simulink model "sf_edge_detection_pulse"  (R2025b)
settings: Solver=FixedStepDiscrete  StartTime=0.0  StopTime=8  FixedStep=1  RelTol=1e-3  EnableMultiTasking=on
settings Model: Creator=The MathWorks, Inc.  LastModifiedBy=The MathWorks, Inc.
settings SolverCC: AlgebraicLoopSolver=TrustRegion  MaxZcPerStep=1.0
settings DataIOCC: LimitDataPoints=on  SaveFormat=Array  ReturnWorkspaceOutputs=off
settings OptimizationCC: ReuseModelBlockBuffer=off  ExpressionDepthLimit=2147483647.0  InitFltsAndDblsToZero=on  LifeSpan=inf
settings DebuggingCC: SaveWithParameterizedLinksMsg=none  UnderspecifiedInitializationDetection=Classic  MergeDetectMultiDrivingBlocksExec=none  SignalResolutionControl=TryResolveAllWithWarning  SolverPrmCheckMsg=warning  FcnCallInpInsideContextMsg=warning  UnconnectedInputMsg=warning  UnconnectedOutputMsg=warning  UnconnectedLineMsg=warning  StateNameClashWarn=warning  SFUnexpectedBacktrackingDiag=warning  SFNoUnconditionalDefaultTransitionDiag=warning  SFExecutionAtInitializationDiag=none  ArithmeticOperatorsInVariantConditions=warning
settings HardwareCC: ProdBitPerPointer=32.0  ProdBitPerSizeT=32.0  ProdBitPerPtrDiffT=32.0  ProdLargestAtomicFloat=None  ProdIntDivRoundTo=Undefined  ProdEndianess=Unspecified  ProdWordSize=32.0  ProdHWDeviceType=32-bit Generic
settings ModelReferenceCC: EnableRefExpFcnMdlSchedulingChecks=on  PropagateSignalLabelsOutOfModel=off
settings SFSimCC: SimUseLocalCustomCode=off  SimParseCustomCode=off  CustomCodeUndefinedFunction=UseInterfaceOnly
settings RTWCC: RTWUseLocalCustomCode=off  GPUComputeCapability=3.5  DLArmComputeVersion=19.05
settings CodeAppCC: StateflowObjectComments=on
settings GRTTargetCC: TargetFcnLib=ansi_tfl_tmw.mat  TargetLangStandard=C89/C90 (ANSI)  CombineOutputUpdateFcns=off  GRTInterface=on
settings ConfigComp: CovMetricSettings=dw  CovSaveCumulativeToWorkspaceVar=on  CovSaveSingleToWorkspaceVar=on  CovExternalEMLEnable=off

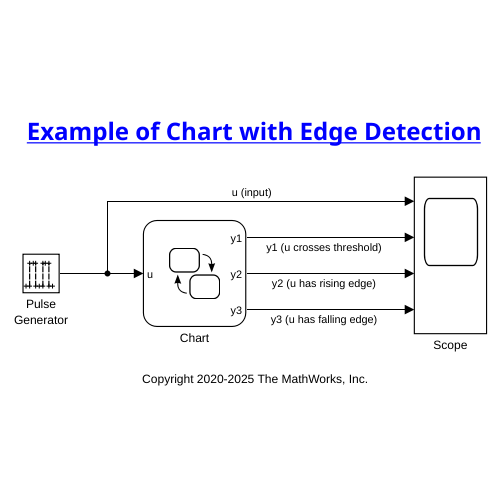
[thumbnail: Simulink's stored preview of the top-level diagram]
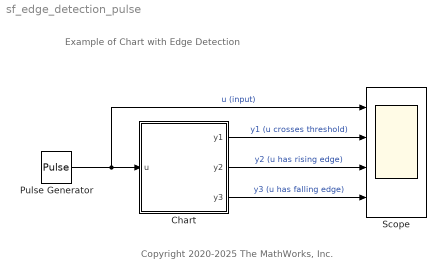
== system sf_edge_detection_pulse ==
  note: Copyright 2020-2025 The MathWorks, Inc.
  note: Example of Chart with Edge Detection
  Chart : Stateflow chart  TreatAsAtomicUnit=on
  Pulse Generator : DiscretePulseGenerator  Amplitude=5  Period=4  PulseWidth=2  PhaseDelay=1
  Scope : Scope  NumInputPorts=4
      settings: ActiveDisplayYMinimum=-0.625  ActiveDisplayYMaximum=5.625
  wires:
  Pulse Generator/1 -> Scope/1, Chart/1(u)  "u (input)"
  Chart/1(y1) -> Scope/2  "y1 (u crosses threshold)"
  Chart/2(y2) -> Scope/3  "y2 (u has rising edge)"
  Chart/3(y3) -> Scope/4  "y3 (u has falling edge)"

== stateflow chart sf_edge_detection_pulse/Chart ==
  (default) -> (junction 2) : {
      | y1 = crossing(u-2.5);
      | y2 = rising(u-2.5);
      | y3 = falling(u-2.5);
      | }
  data: u input double; y1 output boolean; y2 output boolean; y3 output boolean
